simulink model "chaine_filtres"  (R2023b)
settings: Solver=FixedStepDiscrete  StartTime=0.0  StopTime=Tsim  RelTol=1e-3
values from neighbouring files (symbols this model uses):
  d_ech = 1    [parametres_chaine.m]    (also in partie3_q12.m = d)
  graine = 1    [extension_source_huffman.m]    (also in mes_parametres.m = mod(sum(c .* (1:numel(c)) * 31) + 7 * numel(c), 2^31 - 1); parametres_chaine.m = P.graine; parametres_perso.m = mod(sum(c .* (1:numel(c)) * 31) + 7 * numel(c), 2^31 - 1); partie4_q10.m = P.graine)
  h = h / sqrt(sum(h.^2))    [coef_rrc.m]    (also in construire_chaine_base.m = cellfun(@(n) get_param(b(n), 'Handle'), groupes{i, 2}); construire_chaine_codee.m = cellfun(@(n) get_param(b(n), 'Handle'), groupes{i, 2}); construire_chaine_qpsk.m = cellfun(@(n) get_param(b(n), 'Handle'), groupes{i, 2}); construire_chaine_qpsk_codee.m = cellfun(@(n) get_param(b(n), 'Handle'), groupes{i, 2}))
  L = cell(0, 2)    [construire_chaine_qpsk.m]    (also in construire_chaine_qpsk_codee.m; construire_chaine_texte.m; construire_decodeur_hamming.m = {'Mot recu/1', 'Bits r/1'; parametres.m = P.L)
  p1 = P.p1    [parametres.m]    (also in parametres_chaine.m = 0.5; partie3_q4.m; partie3_q5.m; partie3_q8.m = 0.3)
  sigma2 = N0 * L / (2 * Tb)    [parametres_chaine.m]    (also in partie3_q12.m; partie4_q10.m)
  tabB1 = [0 0 1 1]    [partie5_q2.m]    (also in partie5_q3.m; partie5_q4.m; partie5_q5.m = M(m).tabB1)
  tabB2 = [0 1 0 1]    [partie5_q2.m]    (also in partie5_q3.m; partie5_q4.m; partie5_q5.m = M(m).tabB2)
  tabI = [ 1  1 -1 -1] / sqrt(2)    [partie5_q2.m]    (also in partie5_q3.m = [1 1 -1 -1] / sqrt(2); partie5_q4.m = [1 1 -1 -1] / sqrt(2); partie5_q5.m = M(m).tabI)
  tabQ = [ 1 -1  1 -1] / sqrt(2)    [partie5_q2.m]    (also in partie5_q3.m = [1 -1 1 -1] / sqrt(2); partie5_q4.m = [1 -1 1 -1] / sqrt(2); partie5_q5.m = M(m).tabQ)
  Tb = 1    [parametres.m]    (also in parametres_chaine.m; partie3_simulation.m; partie4_q10.m = 7; partie5_q2.m)
  Te = Tb / L    [parametres.m]    (also in parametres_chaine.m; partie3_simulation.m)
  Ts = 2 * Tb    (= 2)    [partie5_q2.m]    (also in partie5_q3.m; partie5_q4.m; partie5_q5.m)
libraries: simulink x6
settings Model: Creator=e2604176  LastModifiedBy=e2604176
settings OptimizationCC: BooleanDataType=off

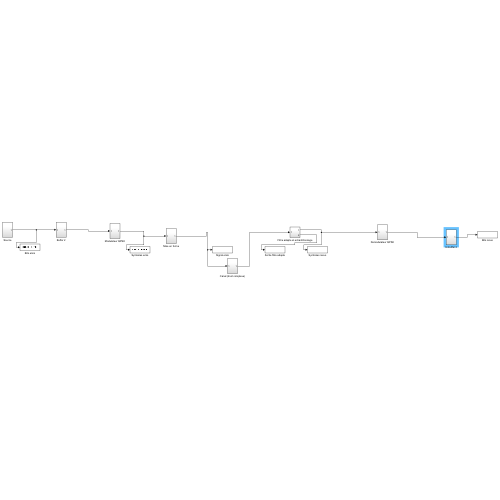
[thumbnail: Simulink's stored preview of the top-level diagram]
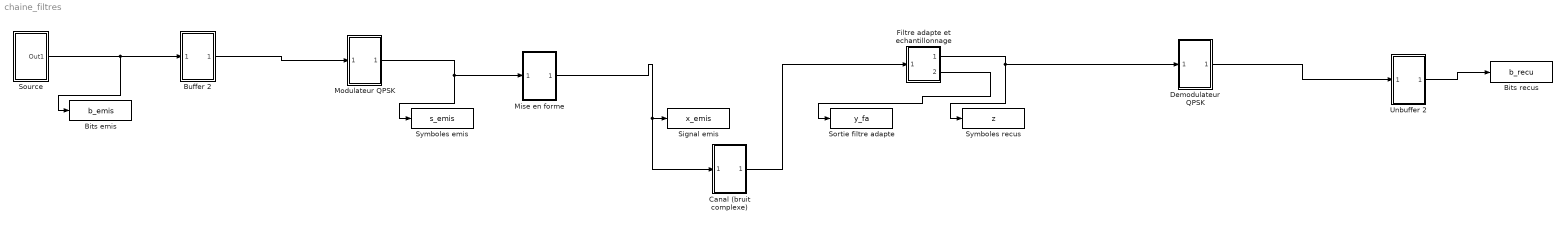
== system chaine_filtres ==
  Bits emis : ToWorkspace  VariableName=b_emis  SampleTime=-1
  Bits recus : ToWorkspace  VariableName=b_recu  SampleTime=-1
  Buffer 2 : Subsystem
  Canal (bruit complexe) : Subsystem
  Demodulateur QPSK : Subsystem
  Filtre adapte et echantillonnage : Subsystem
  Mise en forme : Subsystem
  Modulateur QPSK : Subsystem
  Signal emis : ToWorkspace  VariableName=x_emis  SampleTime=-1
  Sortie filtre adapte : ToWorkspace  VariableName=y_fa  SampleTime=-1
  Source : Subsystem
  Symboles emis : ToWorkspace  VariableName=s_emis  SampleTime=-1
  Symboles recus : ToWorkspace  VariableName=z  SampleTime=-1
  Unbuffer 2 : Subsystem
  wires:
  Source/1(Out1) -> Buffer 2/1(In1), Bits emis/1
  Modulateur QPSK/1(Out1) -> Mise en forme/1(In1), Symboles emis/1
  Buffer 2/1(Out1) -> Modulateur QPSK/1(In1)
  Mise en forme/1(Out1) -> Canal (bruit complexe)/1(In1), Signal emis/1
  Filtre adapte et echantillonnage/1(Out1) -> Demodulateur QPSK/1(In1), Symboles recus/1
  Canal (bruit complexe)/1(Out1) -> Filtre adapte et echantillonnage/1(In1)
  Filtre adapte et echantillonnage/2(Out2) -> Sortie filtre adapte/1
  Demodulateur QPSK/1(Out1) -> Unbuffer 2/1(In1)
  Unbuffer 2/1(Out1) -> Bits recus/1

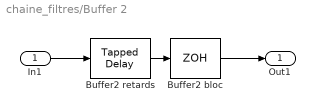
== system chaine_filtres/Buffer 2 ==
  In1 : Inport
  Buffer2 bloc : ZeroOrderHold  SampleTime=Ts
  Buffer2 retards : simulink/Discrete/Tapped Delay  vinit=0  samptime=Tb  NumDelays=1  DelayOrder=Oldest  includeCurrent=on
  Out1 : Outport
  wires:
  Buffer2 retards/1 -> Buffer2 bloc/1
  Buffer2 bloc/1 -> Out1/1
  In1/1 -> Buffer2 retards/1

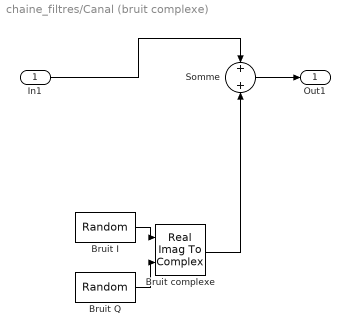
== system chaine_filtres/Canal (bruit complexe) ==
  In1 : Inport
  Bruit I : RandomNumber  Variance=sigma2  Seed=graine + 1  SampleTime=Te
  Bruit Q : RandomNumber  Variance=sigma2  Seed=graine + 2  SampleTime=Te
  Bruit complexe : RealImagToComplex
  Somme : Sum
  Out1 : Outport
  wires:
  Bruit I/1 -> Bruit complexe/1
  Bruit complexe/1 -> Somme/2
  Somme/1 -> Out1/1
  Bruit Q/1 -> Bruit complexe/2
  In1/1 -> Somme/1

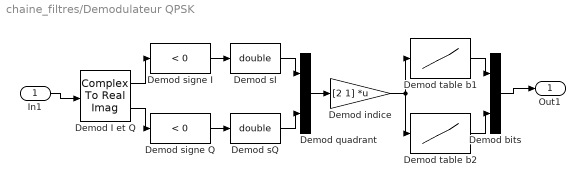
== system chaine_filtres/Demodulateur QPSK ==
  In1 : Inport
  Demod I et Q : ComplexToRealImag
  Demod bits : Mux  Inputs=2
  Demod indice : Gain  Gain=[2 1]  Multiplication=Matrix(K*u)
  Demod quadrant : Mux  Inputs=2
  Demod sI : DataTypeConversion  OutDataTypeStr=double  SaturateOnIntegerOverflow=off  RndMeth=Floor
  Demod sQ : DataTypeConversion  OutDataTypeStr=double  SaturateOnIntegerOverflow=off  RndMeth=Floor
  Demod signe I : simulink/Logic and Bit Operations/Compare To Constant  relop=<  const=0  OutDataTypeStr=boolean
  Demod signe Q : simulink/Logic and Bit Operations/Compare To Constant  relop=<  const=0  OutDataTypeStr=boolean
  Demod table b1 : Lookup_n-D  NumberOfTableDimensions=1  BreakpointsForDimension1=0:3  Table=tabB1  InternalRulePriority=Speed  RndMeth=Simplest
  Demod table b2 : Lookup_n-D  NumberOfTableDimensions=1  BreakpointsForDimension1=0:3  Table=tabB2  InternalRulePriority=Speed  RndMeth=Simplest
  Out1 : Outport
  wires:
  Demod table b2/1 -> Demod bits/2
  In1/1 -> Demod I et Q/1
  Demod I et Q/1 -> Demod signe I/1
  Demod table b1/1 -> Demod bits/1
  Demod sQ/1 -> Demod quadrant/2
  Demod quadrant/1 -> Demod indice/1
  Demod indice/1 -> Demod table b1/1, Demod table b2/1
  Demod signe Q/1 -> Demod sQ/1
  Demod sI/1 -> Demod quadrant/1
  Demod I et Q/2 -> Demod signe Q/1
  Demod signe I/1 -> Demod sI/1
  Demod bits/1 -> Out1/1

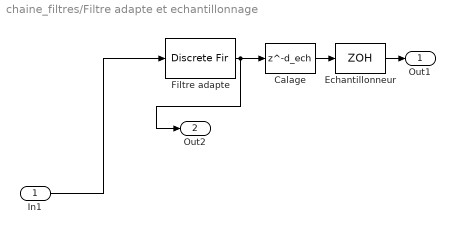
== system chaine_filtres/Filtre adapte et echantillonnage ==
  In1 : Inport
  Calage : Delay  DelayLength=d_ech
  Echantillonneur : ZeroOrderHold  SampleTime=Ts
  Filtre adapte : DiscreteFir  Coefficients=fliplr(h)  SampleTime=Te
  Out1 : Outport
  Out2 : Outport  Port=2
  wires:
  In1/1 -> Filtre adapte/1
  Calage/1 -> Echantillonneur/1
  Filtre adapte/1 -> Out2/1, Calage/1
  Echantillonneur/1 -> Out1/1

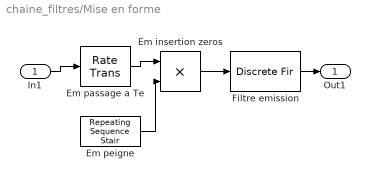
== system chaine_filtres/Mise en forme ==
  In1 : Inport
  Em insertion zeros : Product
  Em passage a Te : RateTransition  OutPortSampleTime=Te
  Em peigne : simulink/Sources/Repeating Sequence Stair  OutValues=[1 zeros(1, L-1)]  tsamp=Te  OutMin=[]  OutMax=[]  OutDataTypeStr=double  OutputDataTypeScalingMode=double  OutDataType=fixdt(0,8)  ConRadixGroup=Best Precision: Vector-wise  OutScaling=2^-12
  Filtre emission : DiscreteFir  Coefficients=h  SampleTime=Te
  Out1 : Outport
  wires:
  Em passage a Te/1 -> Em insertion zeros/1
  Em insertion zeros/1 -> Filtre emission/1
  In1/1 -> Em passage a Te/1
  Em peigne/1 -> Em insertion zeros/2
  Filtre emission/1 -> Out1/1

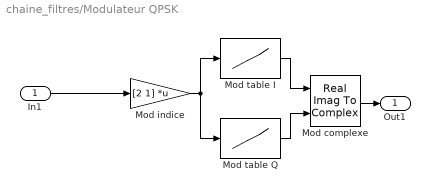
== system chaine_filtres/Modulateur QPSK ==
  In1 : Inport
  Mod complexe : RealImagToComplex
  Mod indice : Gain  Gain=[2 1]  Multiplication=Matrix(K*u)
  Mod table I : Lookup_n-D  NumberOfTableDimensions=1  BreakpointsForDimension1=0:3  Table=tabI  InternalRulePriority=Speed  RndMeth=Simplest
  Mod table Q : Lookup_n-D  NumberOfTableDimensions=1  BreakpointsForDimension1=0:3  Table=tabQ  InternalRulePriority=Speed  RndMeth=Simplest
  Out1 : Outport
  wires:
  Mod table Q/1 -> Mod complexe/2
  Mod indice/1 -> Mod table I/1, Mod table Q/1
  Mod complexe/1 -> Out1/1
  In1/1 -> Mod indice/1
  Mod table I/1 -> Mod complexe/1

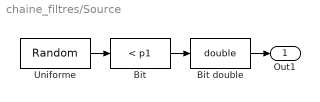
== system chaine_filtres/Source ==
  Bit : simulink/Logic and Bit Operations/Compare To Constant  relop=<  const=p1  OutDataTypeStr=boolean
  Bit double : DataTypeConversion  OutDataTypeStr=double  SaturateOnIntegerOverflow=off  RndMeth=Floor
  Uniforme : UniformRandomNumber  Minimum=0  Seed=graine  SampleTime=Tb
  Out1 : Outport
  wires:
  Bit/1 -> Bit double/1
  Uniforme/1 -> Bit/1
  Bit double/1 -> Out1/1

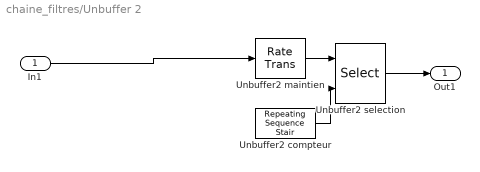
== system chaine_filtres/Unbuffer 2 ==
  In1 : Inport
  Unbuffer2 compteur : simulink/Sources/Repeating Sequence Stair  OutValues=1:2  tsamp=Tb  OutMin=[]  OutMax=[]  OutDataTypeStr=double  OutputDataTypeScalingMode=double  OutDataType=fixdt(0,8)  ConRadixGroup=Best Precision: Vector-wise  OutScaling=2^-12
  Unbuffer2 maintien : RateTransition  OutPortSampleTime=Tb
  Unbuffer2 selection : Selector  InputPortWidth=2  IndexOptions=Index vector (port)  Indices=[1 3]  OutputSizes=1
  Out1 : Outport
  wires:
  Unbuffer2 maintien/1 -> Unbuffer2 selection/1
  Unbuffer2 compteur/1 -> Unbuffer2 selection/2
  Unbuffer2 selection/1 -> Out1/1
  In1/1 -> Unbuffer2 maintien/1
